simulink model "DDMR_Simscape_PID"  (R2024b)
settings: Solver=ode23t  StartTime=0.0  StopTime=30  FixedStep=0.005  RelTol=1e-3
values from neighbouring files (symbols this model uses):
  L = 0.2    [LQR.m]    (also in Track.m; Track2.m)
  L_f = 0.2    [LQR.m]    (also in Track.m; Track2.m)
  line_width = 0.03    [LQR.m]    (also in Track.m; Track2.m)
  N = size(pts, 1)    [Track2.m]
  R = 0.05    [LQR.m]    (also in Track.m; Track2.m)
  track_pts = [2*cos(linspace(0, 2*pi, 1000)'), 2*sin(linspace(0, 2*pi, 1000)').*cos(linspace(0, 2*pi, 1000)')]    [LQR.m]    (also in Track.m; Track2.m = [track_pts; segments{i}])
  W_spread = 0.15    [LQR.m]    (also in Track.m; Track2.m)
undefined symbols (not defined in the file or in its folder): X, Y, Z
libraries: sm_lib x22, nesl_utility x6, slpidlib x2
settings Model: Creator=moham  LastModifiedBy=moham

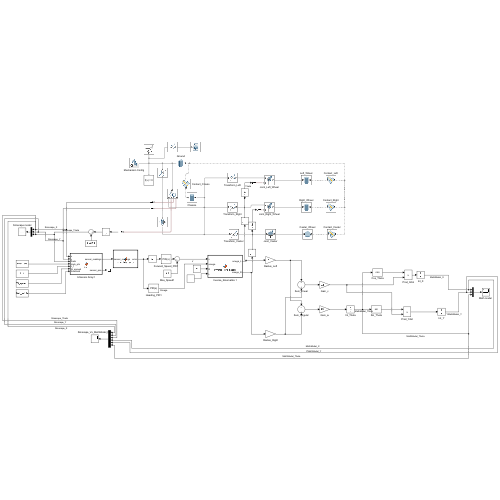
[thumbnail: Simulink's stored preview of the top-level diagram]
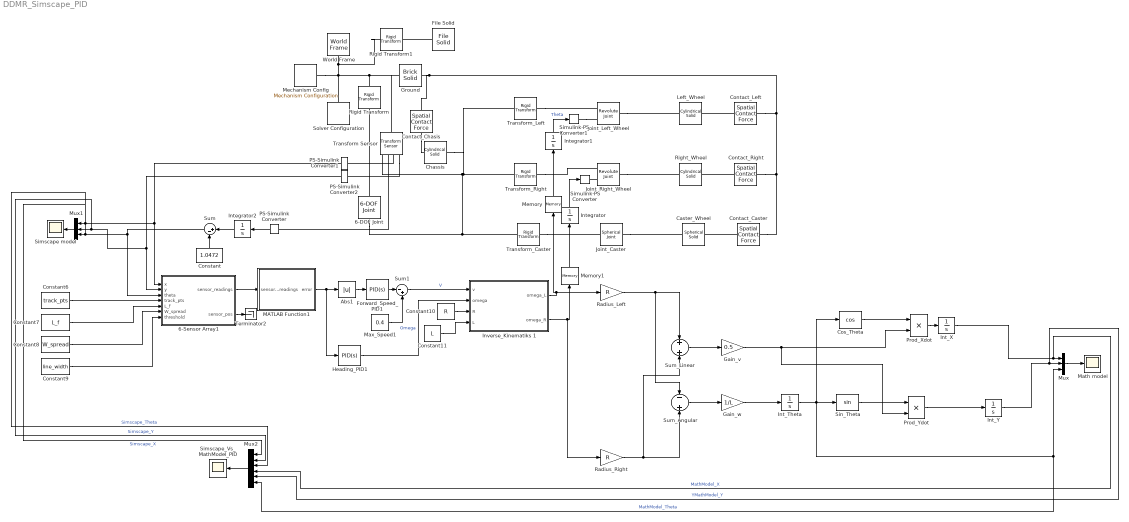
== system DDMR_Simscape_PID ==
  6-DOF Joint : sm_lib/Joints/6-DOF Joint  JointMode=Normal  CompositeWrenchDir=FollowerOnBase  CompositeWrenchFrame=BaseFrame  SenseConstraintForce=off  SenseConstraintTorque=off  SenseTotalForce=off  SenseTotalTorque=off  PxPositionTargetSpecify=off  PxPositionTargetPriority=High  PxPositionTargetValue=0  PxPositionTargetValueUnits=m  PxVelocityTargetSpecify=off  PxVelocityTargetPriority=High  PxVelocityTargetValue=0  PxVelocityTargetValueUnits=m/s  PxEquilibriumPosition=0  PxEquilibriumPositionUnits=m  PxSpringStiffness=0  PxSpringStiffnessUnits=N/m  PxDampingCoefficient=0  PxDampingCoefficientUnits=N/(m/s)  PxLowerLimitSpecify=off  PxLowerLimitBound=-1  PxLowerLimitBoundUnits=m  PxLowerLimitStiffness=1e6  PxLowerLimitStiffnessUnits=N/m  PxLowerLimitDamping=1e3  PxLowerLimitDampingUnits=N/(m/s)  PxLowerLimitTransitionRegionWidth=1e-4  PxLowerLimitTransitionRegionWidthUnits=m  PxUpperLimitSpecify=off  PxUpperLimitBound=1  PxUpperLimitBoundUnits=m  PxUpperLimitStiffness=1e6  PxUpperLimitStiffnessUnits=N/m  PxUpperLimitDamping=1e3  PxUpperLimitDampingUnits=N/(m/s)  PxUpperLimitTransitionRegionWidth=1e-4  PxUpperLimitTransitionRegionWidthUnits=m  PxTorqueActuationMode=NoTorque  PxMotionActuationMode=ComputedMotion  PxSensePosition=off  PxSenseVelocity=off  PxSenseAcceleration=off  PxSenseTorqueForce=off  PxSenseLowerLimitTorqueForce=off  PxSenseUpperLimitTorqueForce=off  PyPositionTargetSpecify=off  PyPositionTargetPriority=High  PyPositionTargetValue=0  PyPositionTargetValueUnits=m  PyVelocityTargetSpecify=off  PyVelocityTargetPriority=High  PyVelocityTargetValue=0  PyVelocityTargetValueUnits=m/s  PyEquilibriumPosition=0  PyEquilibriumPositionUnits=m  PySpringStiffness=0  PySpringStiffnessUnits=N/m  PyDampingCoefficient=0  PyDampingCoefficientUnits=N/(m/s)  PyLowerLimitSpecify=off  PyLowerLimitBound=-1  PyLowerLimitBoundUnits=m  PyLowerLimitStiffness=1e6  PyLowerLimitStiffnessUnits=N/m  PyLowerLimitDamping=1e3  PyLowerLimitDampingUnits=N/(m/s)  PyLowerLimitTransitionRegionWidth=1e-4  PyLowerLimitTransitionRegionWidthUnits=m  PyUpperLimitSpecify=off  PyUpperLimitBound=1  PyUpperLimitBoundUnits=m  PyUpperLimitStiffness=1e6  PyUpperLimitStiffnessUnits=N/m  PyUpperLimitDamping=1e3  PyUpperLimitDampingUnits=N/(m/s)  PyUpperLimitTransitionRegionWidth=1e-4  PyUpperLimitTransitionRegionWidthUnits=m  PyTorqueActuationMode=NoTorque  PyMotionActuationMode=ComputedMotion  PySensePosition=off  PySenseVelocity=off  PySenseAcceleration=off  PySenseTorqueForce=off  PySenseLowerLimitTorqueForce=off  PySenseUpperLimitTorqueForce=off  PzPositionTargetSpecify=on  PzPositionTargetPriority=High  PzPositionTargetValue=0.08  PzPositionTargetValueUnits=m  PzVelocityTargetSpecify=off  PzVelocityTargetPriority=High  PzVelocityTargetValue=0  PzVelocityTargetValueUnits=m/s  PzEquilibriumPosition=0  PzEquilibriumPositionUnits=m  PzSpringStiffness=0  PzSpringStiffnessUnits=N/m  PzDampingCoefficient=0  PzDampingCoefficientUnits=N/(m/s)  PzLowerLimitSpecify=off  PzLowerLimitBound=-1  PzLowerLimitBoundUnits=m  PzLowerLimitStiffness=1e6  PzLowerLimitStiffnessUnits=N/m  PzLowerLimitDamping=1e3  PzLowerLimitDampingUnits=N/(m/s)  PzLowerLimitTransitionRegionWidth=1e-4  PzLowerLimitTransitionRegionWidthUnits=m  PzUpperLimitSpecify=off  PzUpperLimitBound=1  PzUpperLimitBoundUnits=m  PzUpperLimitStiffness=1e6  PzUpperLimitStiffnessUnits=N/m  PzUpperLimitDamping=1e3  PzUpperLimitDampingUnits=N/(m/s)  PzUpperLimitTransitionRegionWidth=1e-4  PzUpperLimitTransitionRegionWidthUnits=m  PzTorqueActuationMode=NoTorque  PzMotionActuationMode=ComputedMotion  PzSensePosition=off  PzSenseVelocity=off  PzSenseAcceleration=off  PzSenseTorqueForce=off  PzSenseLowerLimitTorqueForce=off  PzSenseUpperLimitTorqueForce=off  SphPositionTargetSpecify=off  SphPositionTargetPriority=High  SphPositionTargetRotationMethod=None  SphPositionTargetFollAlignAxisA=+X  SphPositionTargetBaseAlignAxisA=+Y  SphPositionTargetFollAlignAxisB=+Y  SphPositionTargetBaseAlignAxisB=+Z  SphPositionTargetRotationStandardAxis=+Z  SphPositionTargetRotationAngle=0  SphPositionTargetRotationAngleUnits=deg  SphPositionTargetRotationArbitraryAxis=[0 0 1]  SphPositionTargetRotationSequenceAxes=FollowerAxes  SphPositionTargetRotationSequence=XYX  SphPositionTargetRotationSequenceAngles=[0 0 0]  SphPositionTargetRotationSequenceAnglesUnits=deg  SphPositionTargetRotationMatrix=[1 0 0;0 1 0;0 0 1]  SphPositionTargetQuaternion=[1 0 0 0]  SphVelocityTargetSpecify=off  SphVelocityTargetPriority=High  SphVelocityTargetValue=[0 0 0]  SphVelocityTargetValueUnits=deg/s  SphVelocityTargetInFollowerFrame=on  SphEqPosRotationMethod=None  SphEqPosFollAlignAxisA=+X  SphEqPosBaseAlignAxisA=+Y  SphEqPosFollAlignAxisB=+Y  SphEqPosBaseAlignAxisB=+Z  SphEqPosRotationStandardAxis=+Z  SphEqPosRotationAngle=0  SphEqPosRotationAngleUnits=deg  SphEqPosRotationArbitraryAxis=[0 0 1]  SphEqPosRotationSequenceAxes=FollowerAxes  SphEqPosRotationSequence=XYX  SphEqPosRotationSequenceAngles=[0 0 0]  SphEqPosRotationSequenceAnglesUnits=deg  SphEqPosRotationMatrix=[1 0 0;0 1 0;0 0 1]  SphEqPosQuaternion=[1 0 0 0]  SphSpringStiffness=0  SphSpringStiffnessUnits=N*m/deg  SphDampingCoefficient=0  SphDampingCoefficientUnits=N*m/(deg/s)  SphLowerLimitSpecify=off  SphLowerLimitBound=15  SphLowerLimitBoundUnits=deg  SphLowerLimitStiffness=1e4  SphLowerLimitStiffnessUnits=N*m/deg  SphLowerLimitDamping=10  SphLowerLimitDampingUnits=N*m/(deg/s)  SphLowerLimitTransitionRegionWidth=0.1  SphLowerLimitTransitionRegionWidthUnits=deg  SphUpperLimitSpecify=off  SphUpperLimitBound=45  SphUpperLimitBoundUnits=deg  SphUpperLimitStiffness=1e4  SphUpperLimitStiffnessUnits=N*m/deg  SphUpperLimitDamping=10  SphUpperLimitDampingUnits=N*m/(deg/s)  SphUpperLimitTransitionRegionWidth=0.1  SphUpperLimitTransitionRegionWidthUnits=deg  SphTorqueActuationMode=NoTorque  SphActuateTorqueX=off  SphActuateTorqueY=off  SphActuateTorqueZ=off  SphActuateTorque=off  SphActuationFrame=BaseFrame  SphSensePosition=off  SphSenseVelocityX=off  SphSenseVelocityY=off  SphSenseVelocityZ=off  SphSenseVelocity=off  SphSenseAccelerationX=off  SphSenseAccelerationY=off  SphSenseAccelerationZ=off  SphSenseAcceleration=off  SphSenseLowerLimitTorqueMag=off  SphSenseUpperLimitTorqueMag=off  SphSensingFrame=BaseFrame
  6-Sensor Array1 : MATLAB Function  TreatAsAtomicUnit=on
  Abs1 : Abs  SaturateOnIntegerOverflow=off
  Caster_Wheel : sm_lib/Body Elements/Spherical Solid  SphereRadius=0.030  SphereRadiusUnits=m  ExportEntireGeometry=on  InertiaType=CalculateFromGeometry  BasedOnType=Density  Density=1000  DensityUnits=kg/m^3  Mass=1  MassUnits=kg  CenterOfMass=[0 0 0]  CenterOfMassUnits=m  MomentsOfInertia=[1 1 1]  MomentsOfInertiaUnits=kg*m^2  ProductsOfInertia=[0 0 0]  ProductsOfInertiaUnits=kg*m^2  GraphicType=FromGeometry  MarkerShape=Sphere  MarkerSize=10  GraphicVisPropType=SimpleVisualProperties  GraphicDiffuseColor=[0.6353 0.07843 0.1843]  GraphicOpacity=1  GraphicSpecularColor=[0.5 0.5 0.5 1.0]  GraphicAmbientColor=[0.15 0.15 0.15 1.0]  GraphicEmissiveColor=[0.0 0.0 0.0 1.0]  GraphicShininess=75  DoExposeReferenceFrame=on  SerializedFrames=<Frames/>
  Chassis : sm_lib/Body Elements/Cylindrical Solid  CylinderRadius=0.22  CylinderRadiusUnits=m  CylinderLength=5  CylinderLengthUnits=cm  ExportEntireGeometry=on  InertiaType=CalculateFromGeometry  BasedOnType=Mass  Density=1000  DensityUnits=kg/m^3  Mass=5  MassUnits=kg  CenterOfMass=[0 0 0]  CenterOfMassUnits=m  MomentsOfInertia=[1 1 1]  MomentsOfInertiaUnits=kg*m^2  ProductsOfInertia=[0 0 0]  ProductsOfInertiaUnits=kg*m^2  GraphicType=FromGeometry  MarkerShape=Sphere  MarkerSize=10  GraphicVisPropType=SimpleVisualProperties  GraphicDiffuseColor=[0 0.4471 0.7412]  GraphicOpacity=0.5  GraphicSpecularColor=[0.5 0.5 0.5 1.0]  GraphicAmbientColor=[0.15 0.15 0.15 1.0]  GraphicEmissiveColor=[0.0 0.0 0.0 1.0]  GraphicShininess=75  DoExposeReferenceFrame=on  SerializedFrames=<Frames/>
  Constant : Constant  Value=1.0472
  Constant10 : Constant  Value=R
  Constant11 : Constant  Value=L
  Constant6 : Constant  Value=track_pts
  Constant7 : Constant  Value=L_f
  Constant8 : Constant  Value=W_spread
  Constant9 : Constant  Value=line_width
  Contact_Caster : sm_lib/Forces and Torques/Spatial Contact Force  NormalForceType=SmoothSpringDamper  NormalStiffness=1e6  NormalStiffnessUnits=N/m  NormalDamping=1e3  NormalDampingUnits=N/(m/s)  NormalTransitionRegionWidth=1e-4  NormalTransitionRegionWidthUnits=m  FrictionType=SmoothStickSlip  CoefficientOfStaticFriction=0.5  CoefficientOfDynamicFriction=0.3  FrictionalCriticalVelocity=1e-3  FrictionalCriticalVelocityUnits=m/s  SenseContactSignal=off  SensePenetrationDepth=off  SenseSeparationDistance=off  SenseNormalForceMagnitude=off  SenseFrictionalForceMagnitude=off  SenseNormalVelocity=off  SenseTangentialVelocity=off  SenseContactBaseRotation=off  SenseContactBaseTranslation=off  SenseContactFollowerRotation=off  SenseContactFollowerTranslation=off  ZeroCrossDetectContactStartAndEnd=off
  Contact_Chasis : sm_lib/Forces and Torques/Spatial Contact Force  NormalForceType=SmoothSpringDamper  NormalStiffness=1e6  NormalStiffnessUnits=N/m  NormalDamping=1e3  NormalDampingUnits=N/(m/s)  NormalTransitionRegionWidth=1e-4  NormalTransitionRegionWidthUnits=m  FrictionType=SmoothStickSlip  CoefficientOfStaticFriction=0.5  CoefficientOfDynamicFriction=0.3  FrictionalCriticalVelocity=1e-3  FrictionalCriticalVelocityUnits=m/s  SenseContactSignal=off  SensePenetrationDepth=off  SenseSeparationDistance=off  SenseNormalForceMagnitude=off  SenseFrictionalForceMagnitude=off  SenseNormalVelocity=off  SenseTangentialVelocity=off  SenseContactBaseRotation=off  SenseContactBaseTranslation=off  SenseContactFollowerRotation=off  SenseContactFollowerTranslation=off  ZeroCrossDetectContactStartAndEnd=off
  Contact_Left : sm_lib/Forces and Torques/Spatial Contact Force  NormalForceType=SmoothSpringDamper  NormalStiffness=1e6  NormalStiffnessUnits=N/m  NormalDamping=1e3  NormalDampingUnits=N/(m/s)  NormalTransitionRegionWidth=1e-4  NormalTransitionRegionWidthUnits=m  FrictionType=SmoothStickSlip  CoefficientOfStaticFriction=0.5  CoefficientOfDynamicFriction=0.3  FrictionalCriticalVelocity=1e-3  FrictionalCriticalVelocityUnits=m/s  SenseContactSignal=off  SensePenetrationDepth=off  SenseSeparationDistance=off  SenseNormalForceMagnitude=off  SenseFrictionalForceMagnitude=off  SenseNormalVelocity=off  SenseTangentialVelocity=off  SenseContactBaseRotation=off  SenseContactBaseTranslation=off  SenseContactFollowerRotation=off  SenseContactFollowerTranslation=off  ZeroCrossDetectContactStartAndEnd=off
  Contact_Right : sm_lib/Forces and Torques/Spatial Contact Force  NormalForceType=SmoothSpringDamper  NormalStiffness=1e6  NormalStiffnessUnits=N/m  NormalDamping=1e3  NormalDampingUnits=N/(m/s)  NormalTransitionRegionWidth=1e-4  NormalTransitionRegionWidthUnits=m  FrictionType=SmoothStickSlip  CoefficientOfStaticFriction=0.5  CoefficientOfDynamicFriction=0.3  FrictionalCriticalVelocity=1e-3  FrictionalCriticalVelocityUnits=m/s  SenseContactSignal=off  SensePenetrationDepth=off  SenseSeparationDistance=off  SenseNormalForceMagnitude=off  SenseFrictionalForceMagnitude=off  SenseNormalVelocity=off  SenseTangentialVelocity=off  SenseContactBaseRotation=off  SenseContactBaseTranslation=off  SenseContactFollowerRotation=off  SenseContactFollowerTranslation=off  ZeroCrossDetectContactStartAndEnd=off
  Cos_Theta : Trigonometry  Operator=cos
  File Solid : sm_lib/Body Elements/File Solid  ExtGeomFileName=black_track.stl  UnitType=Custom  ExtGeomFileUnits=m  StepReaderType=HEX  ExportConvexHullGeometry=off  InertiaType=Custom  BasedOnType=DensityFromFile  Density=1000  DensityUnits=kg/m^3  Mass=0  MassUnits=kg  CenterOfMass=[0 0 0]  CenterOfMassUnits=m  MomentsOfInertia=[1 1 1]  MomentsOfInertiaUnits=kg*m^2  ProductsOfInertia=[0 0 0]  ProductsOfInertiaUnits=kg*m^2  GraphicType=FromGeometry  MarkerShape=Sphere  MarkerSize=10  GraphicVisPropType=SimpleVisualProperties  GraphicDiffuseColor=[0.149 0.149 0.149]  GraphicOpacity=1  GraphicSpecularColor=[0.5 0.5 0.5 1.0]  GraphicAmbientColor=[0.15 0.15 0.15 1.0]  GraphicEmissiveColor=[0.0 0.0 0.0 1.0]  GraphicShininess=75  DoExposeReferenceFrame=on  SerializedFrames=<Frames/>
  Forward_Speed_PID1 : slpidlib/PID Controller  Controller=PID  Form=Parallel  TimeDomain=Continuous-time  UseExternalTs=off  SampleTime=-1  IntegratorMethod=Forward Euler  FilterMethod=Forward Euler  ControllerParametersSource=internal  P=0.05  I=0  UseKiTs=off  D=0  UseExternalDerivativeSource=off  N=100  UseFilter=on  TunerSelectOption=Transfer Function Based (PID Tuner App)  InitialConditionSource=internal  InitialConditionForIntegrator=0  InitialConditionForFilter=0  DifferentiatorICPrevScaledInput=0  ExternalReset=none  TrackingMode=off  Kt=1  LimitOutput=off  SatLimitsSource=internal  UpperSaturationLimit=inf  LowerSaturationLimit=-inf  LinearizeAsGain=on  AntiWindupMode=none  Kb=1  LimitIntegrator=off  UpperIntegratorSaturationLimit=inf  LowerIntegratorSaturationLimit=-inf  POutMin=[]  POutMax=[]  IOutMin=[]  IOutMax=[]  DOutMin=[]  DOutMax=[]  NOutMin=[]  NOutMax=[]  SumOutMin=[]  SumOutMax=[]  SaturationOutMin=[]  SaturationOutMax=[]  PParamMin=[]  PParamMax=[]  IParamMin=[]  IParamMax=[]  DParamMin=[]  DParamMax=[]  NParamMin=[]  NParamMax=[]  KbParamMin=[]  KbParamMax=[]  KtParamMin=[]  KtParamMax=[]  KbOutMin=[]  KbOutMax=[]  KtOutMin=[]  KtOutMax=[]  IntegratorOutMin=[]  IntegratorOutMax=[]  FilterOutMin=[]  FilterOutMax=[]  SumI1OutMin=[]  SumI1OutMax=[]  SumI2OutMin=[]  SumI2OutMax=[]  SumI3OutMin=[]  SumI3OutMax=[]  SumI4OutMin=[]  SumI4OutMax=[]  SumDOutMin=[]  SumDOutMax=[]  DifferentiatorOutMin=[]  DifferentiatorOutMax=[]  FilterDiffOutCoefMin=[]  FilterDiffOutCoefMax=[]  ReciprocalOutMin=[]  ReciprocalOutMax=[]  SumDenOutMin=[]  SumDenOutMax=[]  SumNumOutMin=[]  SumNumOutMax=[]  DivideOutMin=[]  DivideOutMax=[]  UdiffTsProdOutMin=[]  UdiffTsProdOutMax=[]  NTsProdOutMin=[]  NTsProdOutMax=[]  UintegralTsProdOutMin=[]  UintegralTsProdOutMax=[]  UngainTsProdOutMin=[]  UngainTsProdOutMax=[]  ClampingZeroOutDataTypeStr=Inherit: Inherit via back propagation  ClampingZeroOutMin=[]  ClampingZeroOutMax=[]  FilterDenConstantOutDataTypeStr=Inherit: Inherit via back propagation  FilterDenConstantOutMin=[]  FilterDenConstantOutMax=[]  PCopyOutDataTypeStr=Inherit: Inherit via back propagation  PCopyOutMin=[]  PCopyOutMax=[]  NCopyOutDataTypeStr=Inherit: Inherit via back propagation  NCopyOutMin=[]  NCopyOutMax=[]  IntegratorContinuousStateAttributes=''  IntegratorStateMustResolveToSignalObject=off  IntegratorRTWStateStorageClass=Auto  FilterContinuousStateAttributes=''  FilterStateMustResolveToSignalObject=off  FilterRTWStateStorageClass=Auto  ParallelPVariant=InternalParameters  IdealPVariant=Disabled  IVariant=InternalParameters  DVariant=InternalParameters  IntegratorVariant=Continuous  SatVariant=Disabled  AWVariant=Passthrough  PCopyVariant=Disabled  TRVariant=Disabled  FdbkBlocksVariant=Forward  IdealPFdbkVariant=Disabled  SatFdbkVariant=Disabled  DerivativeFilterVariant=ContFilter  NVariant=InternalParameters  NCopyVariant=Disabled  FilterICVariant=InternalICsFilter  IntegratorICVariant=InternalICs  ExternalResetVariant=Disabled  TRSumVariant=Passthrough  SumFdbkVariant=Disabled  SumVariant=Sum_PID  TsampFilterVariant=InternalTs  TsampNgainVariant=Passthrough  TsampIntegralVariant=Disabled_SignalSpec  ExternalSaturationOutDataTypeStr=Inherit: Same as second input  DerivativeSourceVariant=ErrorSignal  PreIntVariant=InternalPreInt
  Gain_v : Gain  Gain=0.5
  Gain_w : Gain  Gain=1/L
  Ground : sm_lib/Body Elements/Brick Solid  BrickDimensions=[20 20 0.01]  BrickDimensionsUnits=m  ExportEntireGeometry=on  InertiaType=CalculateFromGeometry  BasedOnType=Density  Density=1000  DensityUnits=kg/m^3  Mass=1  MassUnits=kg  CenterOfMass=[0 0 0]  CenterOfMassUnits=m  MomentsOfInertia=[1 1 1]  MomentsOfInertiaUnits=kg*m^2  ProductsOfInertia=[0 0 0]  ProductsOfInertiaUnits=kg*m^2  GraphicType=FromGeometry  MarkerShape=Sphere  MarkerSize=10  GraphicVisPropType=SimpleVisualProperties  GraphicDiffuseColor=[1 1 1]  GraphicOpacity=1  GraphicSpecularColor=[0.5 0.5 0.5 1.0]  GraphicAmbientColor=[0.15 0.15 0.15 1.0]  GraphicEmissiveColor=[0.0 0.0 0.0 1.0]  GraphicShininess=75  DoExposeReferenceFrame=on  SerializedFrames=<Frames/>
  Heading_PID1 : slpidlib/PID Controller  Controller=PID  Form=Parallel  TimeDomain=Continuous-time  UseExternalTs=off  SampleTime=-1  IntegratorMethod=Forward Euler  FilterMethod=Forward Euler  ControllerParametersSource=internal  P=0.167  I=0.0001  UseKiTs=off  D=0.009  UseExternalDerivativeSource=off  N=100  UseFilter=on  TunerSelectOption=Transfer Function Based (PID Tuner App)  InitialConditionSource=internal  InitialConditionForIntegrator=0  InitialConditionForFilter=0  DifferentiatorICPrevScaledInput=0  ExternalReset=none  TrackingMode=off  Kt=1  LimitOutput=off  SatLimitsSource=internal  UpperSaturationLimit=inf  LowerSaturationLimit=-inf  LinearizeAsGain=on  AntiWindupMode=none  Kb=1  LimitIntegrator=off  UpperIntegratorSaturationLimit=inf  LowerIntegratorSaturationLimit=-inf  POutMin=[]  POutMax=[]  IOutMin=[]  IOutMax=[]  DOutMin=[]  DOutMax=[]  NOutMin=[]  NOutMax=[]  SumOutMin=[]  SumOutMax=[]  SaturationOutMin=[]  SaturationOutMax=[]  PParamMin=[]  PParamMax=[]  IParamMin=[]  IParamMax=[]  DParamMin=[]  DParamMax=[]  NParamMin=[]  NParamMax=[]  KbParamMin=[]  KbParamMax=[]  KtParamMin=[]  KtParamMax=[]  KbOutMin=[]  KbOutMax=[]  KtOutMin=[]  KtOutMax=[]  IntegratorOutMin=[]  IntegratorOutMax=[]  FilterOutMin=[]  FilterOutMax=[]  SumI1OutMin=[]  SumI1OutMax=[]  SumI2OutMin=[]  SumI2OutMax=[]  SumI3OutMin=[]  SumI3OutMax=[]  SumI4OutMin=[]  SumI4OutMax=[]  SumDOutMin=[]  SumDOutMax=[]  DifferentiatorOutMin=[]  DifferentiatorOutMax=[]  FilterDiffOutCoefMin=[]  FilterDiffOutCoefMax=[]  ReciprocalOutMin=[]  ReciprocalOutMax=[]  SumDenOutMin=[]  SumDenOutMax=[]  SumNumOutMin=[]  SumNumOutMax=[]  DivideOutMin=[]  DivideOutMax=[]  UdiffTsProdOutMin=[]  UdiffTsProdOutMax=[]  NTsProdOutMin=[]  NTsProdOutMax=[]  UintegralTsProdOutMin=[]  UintegralTsProdOutMax=[]  UngainTsProdOutMin=[]  UngainTsProdOutMax=[]  ClampingZeroOutDataTypeStr=Inherit: Inherit via back propagation  ClampingZeroOutMin=[]  ClampingZeroOutMax=[]  FilterDenConstantOutDataTypeStr=Inherit: Inherit via back propagation  FilterDenConstantOutMin=[]  FilterDenConstantOutMax=[]  PCopyOutDataTypeStr=Inherit: Inherit via back propagation  PCopyOutMin=[]  PCopyOutMax=[]  NCopyOutDataTypeStr=Inherit: Inherit via back propagation  NCopyOutMin=[]  NCopyOutMax=[]  IntegratorContinuousStateAttributes=''  IntegratorStateMustResolveToSignalObject=off  IntegratorRTWStateStorageClass=Auto  FilterContinuousStateAttributes=''  FilterStateMustResolveToSignalObject=off  FilterRTWStateStorageClass=Auto  ParallelPVariant=InternalParameters  IdealPVariant=Disabled  IVariant=InternalParameters  DVariant=InternalParameters  IntegratorVariant=Continuous  SatVariant=Disabled  AWVariant=Passthrough  PCopyVariant=Disabled  TRVariant=Disabled  FdbkBlocksVariant=Forward  IdealPFdbkVariant=Disabled  SatFdbkVariant=Disabled  DerivativeFilterVariant=ContFilter  NVariant=InternalParameters  NCopyVariant=Disabled  FilterICVariant=InternalICsFilter  IntegratorICVariant=InternalICs  ExternalResetVariant=Disabled  TRSumVariant=Passthrough  SumFdbkVariant=Disabled  SumVariant=Sum_PID  TsampFilterVariant=InternalTs  TsampNgainVariant=Passthrough  TsampIntegralVariant=Disabled_SignalSpec  ExternalSaturationOutDataTypeStr=Inherit: Same as second input  DerivativeSourceVariant=ErrorSignal  PreIntVariant=InternalPreInt
  Int_Theta : Integrator  InitialCondition=pi/-3
  Int_X : Integrator
  Int_Y : Integrator
  Integrator : Integrator
  Integrator1 : Integrator
  Integrator2 : Integrator
  Inverse_Kinematiks 1 : MATLAB Function  TreatAsAtomicUnit=on
  Joint_Caster : sm_lib/Joints/Spherical Joint  JointMode=Normal  CompositeWrenchDir=FollowerOnBase  CompositeWrenchFrame=BaseFrame  SenseConstraintForce=off  SenseConstraintTorque=off  SenseTotalForce=off  SenseTotalTorque=off  PositionTargetSpecify=off  PositionTargetPriority=High  PositionTargetRotationMethod=None  PositionTargetFollAlignAxisA=+X  PositionTargetBaseAlignAxisA=+Y  PositionTargetFollAlignAxisB=+Y  PositionTargetBaseAlignAxisB=+Z  PositionTargetRotationStandardAxis=+Z  PositionTargetRotationAngle=0  PositionTargetRotationAngleUnits=deg  PositionTargetRotationArbitraryAxis=[0 0 1]  PositionTargetRotationSequenceAxes=FollowerAxes  PositionTargetRotationSequence=XYX  PositionTargetRotationSequenceAngles=[0 0 0]  PositionTargetRotationSequenceAnglesUnits=deg  PositionTargetRotationMatrix=[1 0 0;0 1 0;0 0 1]  PositionTargetQuaternion=[1 0 0 0]  VelocityTargetSpecify=off  VelocityTargetPriority=High  VelocityTargetValue=[0 0 0]  VelocityTargetValueUnits=deg/s  VelocityTargetInFollowerFrame=on  EqPosRotationMethod=None  EqPosFollAlignAxisA=+X  EqPosBaseAlignAxisA=+Y  EqPosFollAlignAxisB=+Y  EqPosBaseAlignAxisB=+Z  EqPosRotationStandardAxis=+Z  EqPosRotationAngle=0  EqPosRotationAngleUnits=deg  EqPosRotationArbitraryAxis=[0 0 1]  EqPosRotationSequenceAxes=FollowerAxes  EqPosRotationSequence=XYX  EqPosRotationSequenceAngles=[0 0 0]  EqPosRotationSequenceAnglesUnits=deg  EqPosRotationMatrix=[1 0 0;0 1 0;0 0 1]  EqPosQuaternion=[1 0 0 0]  SpringStiffness=0  SpringStiffnessUnits=N*m/deg  DampingCoefficient=0  DampingCoefficientUnits=N*m/(deg/s)  LowerLimitSpecify=off  LowerLimitBound=15  LowerLimitBoundUnits=deg  LowerLimitStiffness=1e4  LowerLimitStiffnessUnits=N*m/deg  LowerLimitDamping=10  LowerLimitDampingUnits=N*m/(deg/s)  LowerLimitTransitionRegionWidth=0.1  LowerLimitTransitionRegionWidthUnits=deg  UpperLimitSpecify=off  UpperLimitBound=45  UpperLimitBoundUnits=deg  UpperLimitStiffness=1e4  UpperLimitStiffnessUnits=N*m/deg  UpperLimitDamping=10  UpperLimitDampingUnits=N*m/(deg/s)  UpperLimitTransitionRegionWidth=0.1  UpperLimitTransitionRegionWidthUnits=deg  TorqueActuationMode=NoTorque  ActuateTorqueX=off  ActuateTorqueY=off  ActuateTorqueZ=off  ActuateTorque=off  ActuationFrame=BaseFrame  SensePosition=off  SenseVelocityX=off  SenseVelocityY=off  SenseVelocityZ=off  SenseVelocity=off  SenseAccelerationX=off  SenseAccelerationY=off  SenseAccelerationZ=off  SenseAcceleration=off  SenseLowerLimitTorqueMag=off  SenseUpperLimitTorqueMag=off  SensingFrame=BaseFrame
  Joint_Left_Wheel : sm_lib/Joints/Revolute Joint  JointMode=Normal  CompositeWrenchDir=FollowerOnBase  CompositeWrenchFrame=BaseFrame  SenseConstraintForce=off  SenseConstraintTorque=off  SenseTotalForce=off  SenseTotalTorque=off  PositionTargetSpecify=off  PositionTargetPriority=High  PositionTargetValue=0  PositionTargetValueUnits=deg  VelocityTargetSpecify=off  VelocityTargetPriority=High  VelocityTargetValue=0  VelocityTargetValueUnits=deg/s  EquilibriumPosition=0  EquilibriumPositionUnits=deg  SpringStiffness=0  SpringStiffnessUnits=N*m/deg  DampingCoefficient=0  DampingCoefficientUnits=N*m/(deg/s)  LowerLimitSpecify=off  LowerLimitBound=-90  LowerLimitBoundUnits=deg  LowerLimitStiffness=1e4  LowerLimitStiffnessUnits=N*m/deg  LowerLimitDamping=10  LowerLimitDampingUnits=N*m/(deg/s)  LowerLimitTransitionRegionWidth=0.1  LowerLimitTransitionRegionWidthUnits=deg  UpperLimitSpecify=off  UpperLimitBound=90  UpperLimitBoundUnits=deg  UpperLimitStiffness=1e4  UpperLimitStiffnessUnits=N*m/deg  UpperLimitDamping=10  UpperLimitDampingUnits=N*m/(deg/s)  UpperLimitTransitionRegionWidth=0.1  UpperLimitTransitionRegionWidthUnits=deg  TorqueActuationMode=ComputedTorque  MotionActuationMode=InputMotion  SensePosition=off  SenseVelocity=off  SenseAcceleration=off  SenseTorqueForce=off  SenseLowerLimitTorqueForce=off  SenseUpperLimitTorqueForce=off
  Joint_Right_Wheel : sm_lib/Joints/Revolute Joint  JointMode=Normal  CompositeWrenchDir=FollowerOnBase  CompositeWrenchFrame=BaseFrame  SenseConstraintForce=off  SenseConstraintTorque=off  SenseTotalForce=off  SenseTotalTorque=off  PositionTargetSpecify=off  PositionTargetPriority=High  PositionTargetValue=0  PositionTargetValueUnits=deg  VelocityTargetSpecify=off  VelocityTargetPriority=High  VelocityTargetValue=0  VelocityTargetValueUnits=deg/s  EquilibriumPosition=0  EquilibriumPositionUnits=deg  SpringStiffness=0  SpringStiffnessUnits=N*m/deg  DampingCoefficient=0  DampingCoefficientUnits=N*m/(deg/s)  LowerLimitSpecify=off  LowerLimitBound=-90  LowerLimitBoundUnits=deg  LowerLimitStiffness=1e4  LowerLimitStiffnessUnits=N*m/deg  LowerLimitDamping=10  LowerLimitDampingUnits=N*m/(deg/s)  LowerLimitTransitionRegionWidth=0.1  LowerLimitTransitionRegionWidthUnits=deg  UpperLimitSpecify=off  UpperLimitBound=90  UpperLimitBoundUnits=deg  UpperLimitStiffness=1e4  UpperLimitStiffnessUnits=N*m/deg  UpperLimitDamping=10  UpperLimitDampingUnits=N*m/(deg/s)  UpperLimitTransitionRegionWidth=0.1  UpperLimitTransitionRegionWidthUnits=deg  TorqueActuationMode=ComputedTorque  MotionActuationMode=InputMotion  SensePosition=off  SenseVelocity=off  SenseAcceleration=off  SenseTorqueForce=off  SenseLowerLimitTorqueForce=off  SenseUpperLimitTorqueForce=off
  Left_Wheel : sm_lib/Body Elements/Cylindrical Solid  CylinderRadius=0.05  CylinderRadiusUnits=m  CylinderLength=0.02  CylinderLengthUnits=m  ExportEntireGeometry=on  InertiaType=CalculateFromGeometry  BasedOnType=Density  Density=1000  DensityUnits=kg/m^3  Mass=1  MassUnits=kg  CenterOfMass=[0 0 0]  CenterOfMassUnits=m  MomentsOfInertia=[1 1 1]  MomentsOfInertiaUnits=kg*m^2  ProductsOfInertia=[0 0 0]  ProductsOfInertiaUnits=kg*m^2  GraphicType=FromGeometry  MarkerShape=Sphere  MarkerSize=10  GraphicVisPropType=SimpleVisualProperties  GraphicDiffuseColor=[0.6353 0.07843 0.1843]  GraphicOpacity=1  GraphicSpecularColor=[0.5 0.5 0.5 1.0]  GraphicAmbientColor=[0.15 0.15 0.15 1.0]  GraphicEmissiveColor=[0.0 0.0 0.0 1.0]  GraphicShininess=75  DoExposeReferenceFrame=on  SerializedFrames=<Frames/>
  MATLAB Function1 : MATLAB Function  TreatAsAtomicUnit=on
  "Math model " : Scope
  Max_Speed1 : Constant  Value=0.4
  Mechanism Config : sm_lib/Utilities/Mechanism Configuration  UniformGravity=Constant  GravityVector=[0 0 -9.80665]  GravityVectorUnits=m/s^2  LinearizationDelta=0.001  JointModeTransitionNonlinearIterations=2
  Memory : Memory
  Memory1 : Memory
  Mux : Mux  Inputs=3
  Mux1 : Mux  Inputs=3
  Mux2 : Mux  Inputs=6
  PS-Simulink Converter : nesl_utility/PS-Simulink Converter  PhysicalDomain=network_engine_domain  SubClassName=ps_output  LeftPortType=input  RightPortType=output  PseudoPeriodic=off  Frequencies=[]  VectorFormat=inherit  Unit=inherit  AffineConversion=off
  PS-Simulink Converter1 : nesl_utility/PS-Simulink Converter  PhysicalDomain=network_engine_domain  SubClassName=ps_output  LeftPortType=input  RightPortType=output  PseudoPeriodic=off  Frequencies=[]  VectorFormat=inherit  Unit=inherit  AffineConversion=off
  PS-Simulink Converter2 : nesl_utility/PS-Simulink Converter  PhysicalDomain=network_engine_domain  SubClassName=ps_output  LeftPortType=input  RightPortType=output  PseudoPeriodic=off  Frequencies=[]  VectorFormat=inherit  Unit=inherit  AffineConversion=off
  Prod_Xdot : Product
  Prod_Ydot : Product
  Radius_Left : Gain  Gain=R
  Radius_Right : Gain  Gain=R
  Right_Wheel : sm_lib/Body Elements/Cylindrical Solid  CylinderRadius=0.05  CylinderRadiusUnits=m  CylinderLength=0.02  CylinderLengthUnits=m  ExportEntireGeometry=on  InertiaType=CalculateFromGeometry  BasedOnType=Density  Density=1000  DensityUnits=kg/m^3  Mass=1  MassUnits=kg  CenterOfMass=[0 0 0]  CenterOfMassUnits=m  MomentsOfInertia=[1 1 1]  MomentsOfInertiaUnits=kg*m^2  ProductsOfInertia=[0 0 0]  ProductsOfInertiaUnits=kg*m^2  GraphicType=FromGeometry  MarkerShape=Sphere  MarkerSize=10  GraphicVisPropType=SimpleVisualProperties  GraphicDiffuseColor=[0.6353 0.07843 0.1843]  GraphicOpacity=1  GraphicSpecularColor=[0.5 0.5 0.5 1.0]  GraphicAmbientColor=[0.15 0.15 0.15 1.0]  GraphicEmissiveColor=[0.0 0.0 0.0 1.0]  GraphicShininess=75  DoExposeReferenceFrame=on  SerializedFrames=<Frames/>
  Rigid Transform : sm_lib/Frames and Transforms/Rigid Transform  RotationMethod=StandardAxis  FollAlignAxisA=+X  BaseAlignAxisA=+Y  FollAlignAxisB=+Y  BaseAlignAxisB=+Z  RotationStandardAxis=+Z  RotationAngle=-1.0472  RotationAngleUnits=rad  RotationArbitraryAxis=[0 0 1]  RotationSequenceAxes=FollowerAxes  RotationSequence=XYX  RotationSequenceAngles=[0 0 0]  RotationSequenceAnglesUnits=deg  RotationMatrix=[1 0 0;0 1 0;0 0 1]  Quaternion=[1 0 0 0]  TranslationMethod=None  TranslationCartesianOffset=[0 0 0]  TranslationCartesianOffsetUnits=m  TranslationStandardAxis=+Z  TranslationStandardOffset=0  TranslationStandardOffsetUnits=m  TranslationROffset=0  TranslationROffsetUnits=m  TranslationThetaOffset=0  TranslationThetaOffsetUnits=deg  TranslationZOffset=0  TranslationZOffsetUnits=m
  Rigid Transform1 : sm_lib/Frames and Transforms/Rigid Transform  RotationMethod=None  FollAlignAxisA=+X  BaseAlignAxisA=+Y  FollAlignAxisB=+Y  BaseAlignAxisB=+Z  RotationStandardAxis=+Z  RotationAngle=0  RotationAngleUnits=deg  RotationArbitraryAxis=[0 0 1]  RotationSequenceAxes=FollowerAxes  RotationSequence=XYX  RotationSequenceAngles=[0 0 0]  RotationSequenceAnglesUnits=deg  RotationMatrix=[1 0 0;0 1 0;0 0 1]  Quaternion=[1 0 0 0]  TranslationMethod=StandardAxis  TranslationCartesianOffset=[0 0 0]  TranslationCartesianOffsetUnits=m  TranslationStandardAxis=+Z  TranslationStandardOffset=0.011  TranslationStandardOffsetUnits=m  TranslationROffset=0  TranslationROffsetUnits=m  TranslationThetaOffset=0  TranslationThetaOffsetUnits=deg  TranslationZOffset=0  TranslationZOffsetUnits=m
  Simscape model : Scope
  Simscape_Vs_MathModel_PID : Scope
  Simulink-PS Converter : nesl_utility/Simulink-PS Converter  PhysicalDomain=network_engine_domain  SubClassName=ps_input  LeftPortType=input  RightPortType=output  PseudoPeriodic=off  Frequencies=[]  NoiseDistribution=none  NoiseParameters=[]  Unit=rad  AffineConversion=off  FilteringAndDerivatives=filter  SimscapeFilterOrder=2  InputFilterTimeConstant=0.05  UdotUserProvided=0
  Simulink-PS Converter1 : nesl_utility/Simulink-PS Converter  PhysicalDomain=network_engine_domain  SubClassName=ps_input  LeftPortType=input  RightPortType=output  PseudoPeriodic=off  Frequencies=[]  NoiseDistribution=none  NoiseParameters=[]  Unit=rad  AffineConversion=off  FilteringAndDerivatives=filter  SimscapeFilterOrder=2  InputFilterTimeConstant=0.05  UdotUserProvided=0
  Sin_Theta : Trigonometry
  Solver Configuration : nesl_utility/Solver Configuration  PhysicalDomain=network_engine_domain  SubClassName=solver  LeftPortType=input  RightPortType=generic  Tones=[]  Harmonics=[]  SimulateNoise=off  Profile=off  UseLocalSampling=off  EnableSwitchedLinearOptims=on  FrequencyDomain=off  UseCCode=off  RelTol=0.001  AbsTol=0.001  MinStep=1e-09  ToWorkspace=off  RevertToSquareIcSolve=off  NumHomotopyIterations=100  PhasorMode=off  PhasorModeNumHarmonics=1  ConsistencySolver=NEWTON_XTOL_AFTER_FTOL  IndexReductionMethod=DerivativeReplacement  DoDC=off  ResidualTolerance=1e-09  ConsistencyTolSource=GLOBAL  ConsistencyAbsTol=0.001  ConsistencyRelTol=0.001  ConsistencyTolFactor=0.001  UseLocalSolver=on  LocalSolverChoice=NE_BACKWARD_EULER_ADVANCER  ResolveIndetEquations=on  FunctionEvalNumThread=1  LocalSolverSampleTime=0.005  DoFixedCost=off  MaxNonlinIter=3  MaxModeIter=2  ComputeImpulses=off  ImpulseIterations=2  LinearAlgebra=auto  LinearAlgebraNumThread=0  EquationFormulation=NE_TIME_EF  DelaysMemoryBudget=1024  AutomaticFiltering=on  FilteringTimeConstant=0.001  PartitionStorageMethod=AS_NEEDED  PartitionMemoryBudget=1024  PartitionMethod=ROBUST  MultibodyUseLocalSolver=off  MultibodyLocalSolverChoice=ODE1  MultibodyLocalSolverSampleTime=0.001
  Sum : Sum  Inputs=|+-
  Sum1 : Sum  Inputs=|-+
  Sum_Angular : Sum  Inputs=-+
  Sum_Linear : Sum
  Terminator2 : Terminator
  Transform Sensor : sm_lib/Frames and Transforms/Transform Sensor  MeasurementFrame=World  RotationSequence=XYX  SenseAngle=off  SenseAxis=off  SenseQ=off  SenseR=off  SenseRotationSequence=off  SenseOmegaX=off  SenseOmegaY=off  SenseOmegaZ=on  SenseOmega=off  SenseQDot=off  SenseRDot=off  SenseRotationSequenceDot=off  SenseAlphaX=off  SenseAlphaY=off  SenseAlphaZ=off  SenseAlpha=off  SenseQDDot=off  SenseRDDot=off  SenseX=on  SenseY=on  SenseZ=off  SenseXYZ=off  SenseRad=off  SenseAzim=off  SenseDist=off  SenseInc=off  SenseXDot=off  SenseYDot=off  SenseZDot=off  SenseXYZDot=off  SenseRadDot=off  SenseAzimDot=off  SenseDistDot=off  SenseIncDot=off  SenseXDDot=off  SenseYDDot=off  SenseZDDot=off  SenseXYZDDot=off  SenseRadDDot=off  SenseAzimDDot=off  SenseDistDDot=off  SenseIncDDot=off
  Transform_Caster : sm_lib/Frames and Transforms/Rigid Transform  RotationMethod=None  FollAlignAxisA=+X  BaseAlignAxisA=+Y  FollAlignAxisB=+Y  BaseAlignAxisB=+Z  RotationStandardAxis=+Z  RotationAngle=0  RotationAngleUnits=deg  RotationArbitraryAxis=[0 0 1]  RotationSequenceAxes=FollowerAxes  RotationSequence=XYX  RotationSequenceAngles=[0 0 0]  RotationSequenceAnglesUnits=deg  RotationMatrix=[1 0 0;0 1 0;0 0 1]  Quaternion=[1 0 0 0]  TranslationMethod=Cartesian  TranslationCartesianOffset=[0.15, 0, -0.045]  TranslationCartesianOffsetUnits=m  TranslationStandardAxis=+Z  TranslationStandardOffset=0  TranslationStandardOffsetUnits=m  TranslationROffset=0  TranslationROffsetUnits=m  TranslationThetaOffset=0  TranslationThetaOffsetUnits=deg  TranslationZOffset=0  TranslationZOffsetUnits=m
  Transform_Left : sm_lib/Frames and Transforms/Rigid Transform  RotationMethod=StandardAxis  FollAlignAxisA=+X  BaseAlignAxisA=+Y  FollAlignAxisB=+Y  BaseAlignAxisB=+Z  RotationStandardAxis=+X  RotationAngle=-90  RotationAngleUnits=deg  RotationArbitraryAxis=[0 0 1]  RotationSequenceAxes=FollowerAxes  RotationSequence=XYX  RotationSequenceAngles=[0 0 0]  RotationSequenceAnglesUnits=deg  RotationMatrix=[1 0 0;0 1 0;0 0 1]  Quaternion=[1 0 0 0]  TranslationMethod=Cartesian  TranslationCartesianOffset=[0, 0.1, -0.025]  TranslationCartesianOffsetUnits=m  TranslationStandardAxis=+Z  TranslationStandardOffset=0  TranslationStandardOffsetUnits=m  TranslationROffset=0  TranslationROffsetUnits=m  TranslationThetaOffset=0  TranslationThetaOffsetUnits=deg  TranslationZOffset=0  TranslationZOffsetUnits=m
  Transform_Right : sm_lib/Frames and Transforms/Rigid Transform  RotationMethod=StandardAxis  FollAlignAxisA=+X  BaseAlignAxisA=+Y  FollAlignAxisB=+Y  BaseAlignAxisB=+Z  RotationStandardAxis=+X  RotationAngle=-90  RotationAngleUnits=deg  RotationArbitraryAxis=[0 0 1]  RotationSequenceAxes=FollowerAxes  RotationSequence=XYX  RotationSequenceAngles=[0 0 0]  RotationSequenceAnglesUnits=deg  RotationMatrix=[1 0 0;0 1 0;0 0 1]  Quaternion=[1 0 0 0]  TranslationMethod=Cartesian  TranslationCartesianOffset=[0, -0.1, -0.025]  TranslationCartesianOffsetUnits=m  TranslationStandardAxis=+Z  TranslationStandardOffset=0  TranslationStandardOffsetUnits=m  TranslationROffset=0  TranslationROffsetUnits=m  TranslationThetaOffset=0  TranslationThetaOffsetUnits=deg  TranslationZOffset=0  TranslationZOffsetUnits=m
  World Frame : sm_lib/Frames and Transforms/World Frame
  wires:
  Constant6/1 -> 6-Sensor Array1/4(track_pts)
  Constant11/1 -> Inverse_Kinematiks 1/4(L)
  Forward_Speed_PID1/1 -> Sum1/1
  Max_Speed1/1 -> Sum1/2
  Sum1/1 -> Inverse_Kinematiks 1/1(v)  "V"
  MATLAB Function1/1(error) -> Heading_PID1/1, Abs1/1
  Constant9/1 -> 6-Sensor Array1/7(threshold)
  Constant10/1 -> Inverse_Kinematiks 1/3(R)
  Abs1/1 -> Forward_Speed_PID1/1
  Constant7/1 -> 6-Sensor Array1/5(L_f)
  6-Sensor Array1/1(sensor_readings) -> MATLAB Function1/1(sensor_readings)
  Heading_PID1/1 -> Inverse_Kinematiks 1/2(omega)  "Omega"
  Constant8/1 -> 6-Sensor Array1/6(W_spread)
  6-Sensor Array1/2(sensor_pos) -> Terminator2/1
  Memory/1 -> Integrator1/1
  Memory1/1 -> Integrator/1
  Inverse_Kinematiks 1/2(omega_R) -> Radius_Right/1, Memory1/1
  Prod_Ydot/1 -> Int_Y/1
  Prod_Xdot/1 -> Int_X/1
  Int_Theta/1 -> Cos_Theta/1, Mux/3, Mux2/6, Sin_Theta/1  "MathModel_Theta"
  Sum_Linear/1 -> Gain_v/1
  Gain_w/1 -> Int_Theta/1
  Radius_Left/1 -> Sum_Linear/1, Sum_Angular/1
  Sin_Theta/1 -> Prod_Ydot/1
  Cos_Theta/1 -> Prod_Xdot/1
  Sum_Angular/1 -> Gain_w/1
  Gain_v/1 -> Prod_Xdot/2, Prod_Ydot/2
  Inverse_Kinematiks 1/1(omega_L) -> Radius_Left/1, Memory/1
  Radius_Right/1 -> Sum_Linear/2, Sum_Angular/2
  Mux/1 -> "Math model "/1
  Int_X/1 -> Mux2/4, Mux/1  "MathModel_X"
  Int_Y/1 -> Mux/2, Mux2/5  "YMathModel_Y"
  Mux1/1 -> Simscape model/1
  Integrator1/1 -> Simulink-PS Converter1/1  "Theta"
  Integrator/1 -> Simulink-PS Converter/1
  PS-Simulink Converter/1 -> Integrator2/1
  Integrator2/1 -> Sum/1
  Constant/1 -> Sum/2
  Sum/1 -> 6-Sensor Array1/3(theta), Mux2/3, Mux1/3  "Simscape_Theta"
  PS-Simulink Converter2/1 -> Mux1/2, Mux2/2, 6-Sensor Array1/2(y)  "Simscape_Y"
  PS-Simulink Converter1/1 -> Mux2/1, Mux1/1, 6-Sensor Array1/1(x)  "Simscape_X"
  Mux2/1 -> Simscape_Vs_MathModel_PID/1
  connections:
  Contact_Caster/LConn1 -- Contact_Right/LConn1 -- Contact_Left/LConn1 -- Contact_Chasis/RConn1 -- Ground/LConn1
  Solver Configuration/RConn1 -- Transform Sensor/LConn1 -- Ground/RConn1 -- Rigid Transform/LConn1 -- Rigid Transform1/LConn1 -- World Frame/RConn1 -- Mechanism Config/RConn1
  Transform_Caster/LConn1 -- 6-DOF Joint/RConn1 -- Chassis/RConn1 -- Transform_Left/LConn1 -- Transform_Right/LConn1 -- Transform Sensor/RConn1
  Transform_Right/RConn1 -- Joint_Right_Wheel/LConn1
  Transform_Caster/RConn1 -- Joint_Caster/LConn1
  Contact_Left/RConn1 -- Left_Wheel/LConn1
  Joint_Left_Wheel/RConn1 -- Left_Wheel/RConn1
  Joint_Caster/RConn1 -- Caster_Wheel/RConn1
  Contact_Right/RConn1 -- Right_Wheel/LConn1
  Joint_Right_Wheel/RConn1 -- Right_Wheel/RConn1
  Contact_Caster/RConn1 -- Caster_Wheel/LConn1
  Transform_Left/RConn1 -- Joint_Left_Wheel/LConn1
  Simulink-PS Converter/RConn1 -- Joint_Right_Wheel/LConn2
  Simulink-PS Converter1/RConn1 -- Joint_Left_Wheel/LConn2
  File Solid/RConn1 -- Rigid Transform1/RConn1
  Transform Sensor/RConn2 -- PS-Simulink Converter/LConn1
  Transform Sensor/RConn3 -- PS-Simulink Converter1/LConn1
  Transform Sensor/RConn4 -- PS-Simulink Converter2/LConn1
  6-DOF Joint/LConn1 -- Rigid Transform/RConn1
  Contact_Chasis/LConn1 -- Chassis/LConn1

== matlab function DDMR_Simscape_PID/6-Sensor Array1 ==
  data: x input; sensor_readings output; y input; theta input; track_pts input; L_f input; W_spread input; threshold input; sensor_pos output
function [sensor_readings, sensor_pos] = fcn(x, y, theta, track_pts, L_f, W_spread, threshold)
    % 6 sensors spread linearly across the front
    y_offsets = linspace(W_spread/2, -W_spread/2, 6);
    S_loc = [L_f * ones(1,6); y_offsets];
    
    R = [cos(theta), -sin(theta); sin(theta), cos(theta)];
    
    sensor_pos = zeros(2, 6);
    sensor_readings = zeros(1, 6);
    
    for i = 1:6
        % Calculate global position of each sensor
        sensor_pos(:, i) = [x; y] + R * S_loc(:, i);
        
        % Check distance to the track
        dists = sqrt((track_pts(:,1) - sensor_pos(1, i)).^2 + (track_pts(:,2) - sensor_pos(2, i)).^2);
        if min(dists) <= threshold
            sensor_readings(i) = 1;
        end
    end
end

== matlab function DDMR_Simscape_PID/Inverse_Kinematiks 1 ==
  data: v input; omega_L output; omega input; R input; L input; omega_R output
function [omega_L, omega_R] = inverse_kinematics(v, omega, R, L)
    % Calculate linear velocity of each wheel (m/s)
    v_L = v - (omega * L / 2);
    v_R = v + (omega * L / 2);

    % Convert linear velocity to angular velocity (rad/s)
    omega_L = v_L / R;
    omega_R = v_R / R;
end

== matlab function DDMR_Simscape_PID/MATLAB Function1 ==
  settings: updateMethod=DISCRETE
  data: sensor_readings input; error output
function error = calculate_error(sensor_readings)
    % Assign weights to the 6 sensors: far left is positive error, far right is negative
    weights = [5, 3, 1, -1, -3, -5]; 
    
    persistent prev_error;
    if isempty(prev_error)
        prev_error = 0;
    end
    
    if sum(sensor_readings) == 0
        % Track lost: rely on memory to keep steering back toward the line
        error = prev_error; 
    else
        % Track found: calculate new error and update memory
        error = sum(sensor_readings .* weights);
        prev_error = error; 
    end
end
